simulink model "r2_b16a4x64f"  (R2012b)
settings: Solver=VariableStepDiscrete  SolverMode=SingleTasking  StartTime=0.0  StopTime=1  RelTol=1e-3
undefined symbols (not defined in the file): fft_stages, n_bits_ants, n_bits_xengs
libraries: xbsIndex_r4 x26846, casper_library_misc x230, xbsReplacements_r4 x24, casper_library_delays x8, xps_library x5, casper_library_communications x4
(part 19 of 227)

== system r2_b16a4x64f/status2 ==
  out_gbe_down : Inport
  out_rx_dest_err : Inport  Port=2
  out_feng_rx_err : Inport  Port=3
  out_fft_err : Inport  Port=4
  out_feng_qdr_err : Inport  Port=5
  out_feng_chk_err : Inport  Port=6
  out_adc_over : Inport  Port=7
  out_noise_diode_en : Inport  Port=8
  out_vacc_err : Inport  Port=9
  out_rx_bad_pkt : Inport  Port=10
  out_rx_bad_frame : Inport  Port=11
  out_tx_over : Inport  Port=12
  out_xeng_bad_dat : Inport  Port=13
  out_pack_err : Inport  Port=14
  out_rxing_data : Inport  Port=15
  out_txing_data : Inport  Port=16
  out_flushed : Inport  Port=17
  assert_adc_over : xbsIndex_r4/Assert  assert_type=on  type_source=Explicitly  gui_display_data_type=Boolean  arith_type=Boolean  n_bits=1  bin_pt=0  preci_type=Single  exp_width=8  frac_width=24  assert_rate=off  rate_source=Explicitly  period=1  output_port=on  block_type=assert
  assert_feng_chk_err : xbsIndex_r4/Assert  assert_type=on  type_source=Explicitly  gui_display_data_type=Boolean  arith_type=Boolean  n_bits=1  bin_pt=0  preci_type=Single  exp_width=8  frac_width=24  assert_rate=off  rate_source=Explicitly  period=1  output_port=on  block_type=assert
  assert_feng_qdr_err : xbsIndex_r4/Assert  assert_type=on  type_source=Explicitly  gui_display_data_type=Boolean  arith_type=Boolean  n_bits=1  bin_pt=0  preci_type=Single  exp_width=8  frac_width=24  assert_rate=off  rate_source=Explicitly  period=1  output_port=on  block_type=assert
  assert_feng_rx_err : xbsIndex_r4/Assert  assert_type=on  type_source=Explicitly  gui_display_data_type=Boolean  arith_type=Boolean  n_bits=1  bin_pt=0  preci_type=Single  exp_width=8  frac_width=24  assert_rate=off  rate_source=Explicitly  period=1  output_port=on  block_type=assert
  assert_fft_err : xbsIndex_r4/Assert  assert_type=on  type_source=Explicitly  gui_display_data_type=Boolean  arith_type=Boolean  n_bits=1  bin_pt=0  preci_type=Single  exp_width=8  frac_width=24  assert_rate=off  rate_source=Explicitly  period=1  output_port=on  block_type=assert
  assert_flushed : xbsIndex_r4/Assert  assert_type=on  type_source=Explicitly  gui_display_data_type=Boolean  arith_type=Boolean  n_bits=1  bin_pt=0  preci_type=Single  exp_width=8  frac_width=24  assert_rate=off  rate_source=Explicitly  period=1  output_port=on  block_type=assert
  assert_gbe_down : xbsIndex_r4/Assert  assert_type=on  type_source=Explicitly  gui_display_data_type=Boolean  arith_type=Boolean  n_bits=1  bin_pt=0  preci_type=Single  exp_width=8  frac_width=24  assert_rate=off  rate_source=Explicitly  period=1  output_port=on  block_type=assert
  assert_noise_diode_en : xbsIndex_r4/Assert  assert_type=on  type_source=Explicitly  gui_display_data_type=Boolean  arith_type=Boolean  n_bits=1  bin_pt=0  preci_type=Single  exp_width=8  frac_width=24  assert_rate=off  rate_source=Explicitly  period=1  output_port=on  block_type=assert
  assert_pack_err : xbsIndex_r4/Assert  assert_type=on  type_source=Explicitly  gui_display_data_type=Boolean  arith_type=Boolean  n_bits=1  bin_pt=0  preci_type=Single  exp_width=8  frac_width=24  assert_rate=off  rate_source=Explicitly  period=1  output_port=on  block_type=assert
  assert_rx_bad_frame : xbsIndex_r4/Assert  assert_type=on  type_source=Explicitly  gui_display_data_type=Boolean  arith_type=Boolean  n_bits=1  bin_pt=0  preci_type=Single  exp_width=8  frac_width=24  assert_rate=off  rate_source=Explicitly  period=1  output_port=on  block_type=assert
  assert_rx_bad_pkt : xbsIndex_r4/Assert  assert_type=on  type_source=Explicitly  gui_display_data_type=Boolean  arith_type=Boolean  n_bits=1  bin_pt=0  preci_type=Single  exp_width=8  frac_width=24  assert_rate=off  rate_source=Explicitly  period=1  output_port=on  block_type=assert
  assert_rx_dest_err : xbsIndex_r4/Assert  assert_type=on  type_source=Explicitly  gui_display_data_type=Boolean  arith_type=Boolean  n_bits=1  bin_pt=0  preci_type=Single  exp_width=8  frac_width=24  assert_rate=off  rate_source=Explicitly  period=1  output_port=on  block_type=assert
  assert_rxing_data : xbsIndex_r4/Assert  assert_type=on  type_source=Explicitly  gui_display_data_type=Boolean  arith_type=Boolean  n_bits=1  bin_pt=0  preci_type=Single  exp_width=8  frac_width=24  assert_rate=off  rate_source=Explicitly  period=1  output_port=on  block_type=assert
  assert_tx_over : xbsIndex_r4/Assert  assert_type=on  type_source=Explicitly  gui_display_data_type=Boolean  arith_type=Boolean  n_bits=1  bin_pt=0  preci_type=Single  exp_width=8  frac_width=24  assert_rate=off  rate_source=Explicitly  period=1  output_port=on  block_type=assert
  assert_txing_data : xbsIndex_r4/Assert  assert_type=on  type_source=Explicitly  gui_display_data_type=Boolean  arith_type=Boolean  n_bits=1  bin_pt=0  preci_type=Single  exp_width=8  frac_width=24  assert_rate=off  rate_source=Explicitly  period=1  output_port=on  block_type=assert
  assert_vacc_err : xbsIndex_r4/Assert  assert_type=on  type_source=Explicitly  gui_display_data_type=Boolean  arith_type=Boolean  n_bits=1  bin_pt=0  preci_type=Single  exp_width=8  frac_width=24  assert_rate=off  rate_source=Explicitly  period=1  output_port=on  block_type=assert
  assert_xeng_bad_dat : xbsIndex_r4/Assert  assert_type=on  type_source=Explicitly  gui_display_data_type=Boolean  arith_type=Boolean  n_bits=1  bin_pt=0  preci_type=Single  exp_width=8  frac_width=24  assert_rate=off  rate_source=Explicitly  period=1  output_port=on  block_type=assert
  cast_gw : xbsIndex_r4/Convert  gui_display_data_type=Fixed-point  arith_type=Unsigned  n_bits=32  bin_pt=0  float_type=Single  exp_bits=8  fraction_bits=24  quantization=Truncate  overflow=Wrap  en=off  latency=0  dbl_ovrd=off  pipeline=off  block_type=convert
  concatenate : xbsIndex_r4/Concat  num_inputs=17  dbl_ovrd=off  block_type=concat
  io_delay : xbsIndex_r4/Delay  rst=off  infoeditControl=Selection of Reset will increase slice count due to use of real FFs and instead of SRLs  en=off  latency=2  dbl_ovrd=off  reg_retiming=on  block_type=delay
  r2_b16a4x64f_status2_user_data_in : xbsIndex_r4/Gateway Out  inherit_from_input=off  hdl_port=on  timing_constraint=None  locs_specified=off  LOCs={}  UseAsDAC=off  DACChannel='1'  block_type=gatewayout
  reint{1..17} (17 alike) : xbsIndex_r4/Reinterpret  force_arith_type=on  arith_type=Unsigned  force_bin_pt=on  bin_pt=0  block_type=reinterpret
  sim_out : Terminator
  wires:
  concatenate/1 -> io_delay/1
  io_delay/1 -> cast_gw/1
  cast_gw/1 -> r2_b16a4x64f_status2_user_data_in/1
  r2_b16a4x64f_status2_user_data_in/1 -> sim_out/1
  out_gbe_down/1 -> assert_gbe_down/1
  assert_gbe_down/1 -> reint1/1
  reint1/1 -> concatenate/1
  out_rx_dest_err/1 -> assert_rx_dest_err/1
  assert_rx_dest_err/1 -> reint2/1
  reint2/1 -> concatenate/2
  out_feng_rx_err/1 -> assert_feng_rx_err/1
  assert_feng_rx_err/1 -> reint3/1
  reint3/1 -> concatenate/3
  out_fft_err/1 -> assert_fft_err/1
  assert_fft_err/1 -> reint4/1
  reint4/1 -> concatenate/4
  out_feng_qdr_err/1 -> assert_feng_qdr_err/1
  assert_feng_qdr_err/1 -> reint5/1
  reint5/1 -> concatenate/5
  out_feng_chk_err/1 -> assert_feng_chk_err/1
  assert_feng_chk_err/1 -> reint6/1
  reint6/1 -> concatenate/6
  out_adc_over/1 -> assert_adc_over/1
  assert_adc_over/1 -> reint7/1
  reint7/1 -> concatenate/7
  out_noise_diode_en/1 -> assert_noise_diode_en/1
  assert_noise_diode_en/1 -> reint8/1
  reint8/1 -> concatenate/8
  out_vacc_err/1 -> assert_vacc_err/1
  assert_vacc_err/1 -> reint9/1
  reint9/1 -> concatenate/9
  out_rx_bad_pkt/1 -> assert_rx_bad_pkt/1
  assert_rx_bad_pkt/1 -> reint10/1
  reint10/1 -> concatenate/10
  out_rx_bad_frame/1 -> assert_rx_bad_frame/1
  assert_rx_bad_frame/1 -> reint11/1
  reint11/1 -> concatenate/11
  out_tx_over/1 -> assert_tx_over/1
  assert_tx_over/1 -> reint12/1
  reint12/1 -> concatenate/12
  out_xeng_bad_dat/1 -> assert_xeng_bad_dat/1
  assert_xeng_bad_dat/1 -> reint13/1
  reint13/1 -> concatenate/13
  out_pack_err/1 -> assert_pack_err/1
  assert_pack_err/1 -> reint14/1
  reint14/1 -> concatenate/14
  out_rxing_data/1 -> assert_rxing_data/1
  assert_rxing_data/1 -> reint15/1
  reint15/1 -> concatenate/15
  out_txing_data/1 -> assert_txing_data/1
  assert_txing_data/1 -> reint16/1
  reint16/1 -> concatenate/16
  out_flushed/1 -> assert_flushed/1
  assert_flushed/1 -> reint17/1
  reint17/1 -> concatenate/17

== system r2_b16a4x64f/status3 ==
  out_gbe_down : Inport
  out_rx_dest_err : Inport  Port=2
  out_feng_rx_err : Inport  Port=3
  out_fft_err : Inport  Port=4
  out_feng_qdr_err : Inport  Port=5
  out_feng_chk_err : Inport  Port=6
  out_adc_over : Inport  Port=7
  out_noise_diode_en : Inport  Port=8
  out_vacc_err : Inport  Port=9
  out_rx_bad_pkt : Inport  Port=10
  out_rx_bad_frame : Inport  Port=11
  out_tx_over : Inport  Port=12
  out_xeng_bad_dat : Inport  Port=13
  out_pack_err : Inport  Port=14
  out_rxing_data : Inport  Port=15
  out_txing_data : Inport  Port=16
  out_flushed : Inport  Port=17
  assert_adc_over : xbsIndex_r4/Assert  assert_type=on  type_source=Explicitly  gui_display_data_type=Boolean  arith_type=Boolean  n_bits=1  bin_pt=0  preci_type=Single  exp_width=8  frac_width=24  assert_rate=off  rate_source=Explicitly  period=1  output_port=on  block_type=assert
  assert_feng_chk_err : xbsIndex_r4/Assert  assert_type=on  type_source=Explicitly  gui_display_data_type=Boolean  arith_type=Boolean  n_bits=1  bin_pt=0  preci_type=Single  exp_width=8  frac_width=24  assert_rate=off  rate_source=Explicitly  period=1  output_port=on  block_type=assert
  assert_feng_qdr_err : xbsIndex_r4/Assert  assert_type=on  type_source=Explicitly  gui_display_data_type=Boolean  arith_type=Boolean  n_bits=1  bin_pt=0  preci_type=Single  exp_width=8  frac_width=24  assert_rate=off  rate_source=Explicitly  period=1  output_port=on  block_type=assert
  assert_feng_rx_err : xbsIndex_r4/Assert  assert_type=on  type_source=Explicitly  gui_display_data_type=Boolean  arith_type=Boolean  n_bits=1  bin_pt=0  preci_type=Single  exp_width=8  frac_width=24  assert_rate=off  rate_source=Explicitly  period=1  output_port=on  block_type=assert
  assert_fft_err : xbsIndex_r4/Assert  assert_type=on  type_source=Explicitly  gui_display_data_type=Boolean  arith_type=Boolean  n_bits=1  bin_pt=0  preci_type=Single  exp_width=8  frac_width=24  assert_rate=off  rate_source=Explicitly  period=1  output_port=on  block_type=assert
  assert_flushed : xbsIndex_r4/Assert  assert_type=on  type_source=Explicitly  gui_display_data_type=Boolean  arith_type=Boolean  n_bits=1  bin_pt=0  preci_type=Single  exp_width=8  frac_width=24  assert_rate=off  rate_source=Explicitly  period=1  output_port=on  block_type=assert
  assert_gbe_down : xbsIndex_r4/Assert  assert_type=on  type_source=Explicitly  gui_display_data_type=Boolean  arith_type=Boolean  n_bits=1  bin_pt=0  preci_type=Single  exp_width=8  frac_width=24  assert_rate=off  rate_source=Explicitly  period=1  output_port=on  block_type=assert
  assert_noise_diode_en : xbsIndex_r4/Assert  assert_type=on  type_source=Explicitly  gui_display_data_type=Boolean  arith_type=Boolean  n_bits=1  bin_pt=0  preci_type=Single  exp_width=8  frac_width=24  assert_rate=off  rate_source=Explicitly  period=1  output_port=on  block_type=assert
  assert_pack_err : xbsIndex_r4/Assert  assert_type=on  type_source=Explicitly  gui_display_data_type=Boolean  arith_type=Boolean  n_bits=1  bin_pt=0  preci_type=Single  exp_width=8  frac_width=24  assert_rate=off  rate_source=Explicitly  period=1  output_port=on  block_type=assert
  assert_rx_bad_frame : xbsIndex_r4/Assert  assert_type=on  type_source=Explicitly  gui_display_data_type=Boolean  arith_type=Boolean  n_bits=1  bin_pt=0  preci_type=Single  exp_width=8  frac_width=24  assert_rate=off  rate_source=Explicitly  period=1  output_port=on  block_type=assert
  assert_rx_bad_pkt : xbsIndex_r4/Assert  assert_type=on  type_source=Explicitly  gui_display_data_type=Boolean  arith_type=Boolean  n_bits=1  bin_pt=0  preci_type=Single  exp_width=8  frac_width=24  assert_rate=off  rate_source=Explicitly  period=1  output_port=on  block_type=assert
  assert_rx_dest_err : xbsIndex_r4/Assert  assert_type=on  type_source=Explicitly  gui_display_data_type=Boolean  arith_type=Boolean  n_bits=1  bin_pt=0  preci_type=Single  exp_width=8  frac_width=24  assert_rate=off  rate_source=Explicitly  period=1  output_port=on  block_type=assert
  assert_rxing_data : xbsIndex_r4/Assert  assert_type=on  type_source=Explicitly  gui_display_data_type=Boolean  arith_type=Boolean  n_bits=1  bin_pt=0  preci_type=Single  exp_width=8  frac_width=24  assert_rate=off  rate_source=Explicitly  period=1  output_port=on  block_type=assert
  assert_tx_over : xbsIndex_r4/Assert  assert_type=on  type_source=Explicitly  gui_display_data_type=Boolean  arith_type=Boolean  n_bits=1  bin_pt=0  preci_type=Single  exp_width=8  frac_width=24  assert_rate=off  rate_source=Explicitly  period=1  output_port=on  block_type=assert
  assert_txing_data : xbsIndex_r4/Assert  assert_type=on  type_source=Explicitly  gui_display_data_type=Boolean  arith_type=Boolean  n_bits=1  bin_pt=0  preci_type=Single  exp_width=8  frac_width=24  assert_rate=off  rate_source=Explicitly  period=1  output_port=on  block_type=assert
  assert_vacc_err : xbsIndex_r4/Assert  assert_type=on  type_source=Explicitly  gui_display_data_type=Boolean  arith_type=Boolean  n_bits=1  bin_pt=0  preci_type=Single  exp_width=8  frac_width=24  assert_rate=off  rate_source=Explicitly  period=1  output_port=on  block_type=assert
  assert_xeng_bad_dat : xbsIndex_r4/Assert  assert_type=on  type_source=Explicitly  gui_display_data_type=Boolean  arith_type=Boolean  n_bits=1  bin_pt=0  preci_type=Single  exp_width=8  frac_width=24  assert_rate=off  rate_source=Explicitly  period=1  output_port=on  block_type=assert
  cast_gw : xbsIndex_r4/Convert  gui_display_data_type=Fixed-point  arith_type=Unsigned  n_bits=32  bin_pt=0  float_type=Single  exp_bits=8  fraction_bits=24  quantization=Truncate  overflow=Wrap  en=off  latency=0  dbl_ovrd=off  pipeline=off  block_type=convert
  concatenate : xbsIndex_r4/Concat  num_inputs=17  dbl_ovrd=off  block_type=concat
  io_delay : xbsIndex_r4/Delay  rst=off  infoeditControl=Selection of Reset will increase slice count due to use of real FFs and instead of SRLs  en=off  latency=2  dbl_ovrd=off  reg_retiming=on  block_type=delay
  r2_b16a4x64f_status3_user_data_in : xbsIndex_r4/Gateway Out  inherit_from_input=off  hdl_port=on  timing_constraint=None  locs_specified=off  LOCs={}  UseAsDAC=off  DACChannel='1'  block_type=gatewayout
  reint{1..17} (17 alike) : xbsIndex_r4/Reinterpret  force_arith_type=on  arith_type=Unsigned  force_bin_pt=on  bin_pt=0  block_type=reinterpret
  sim_out : Terminator
  wires:
  concatenate/1 -> io_delay/1
  io_delay/1 -> cast_gw/1
  cast_gw/1 -> r2_b16a4x64f_status3_user_data_in/1
  r2_b16a4x64f_status3_user_data_in/1 -> sim_out/1
  out_gbe_down/1 -> assert_gbe_down/1
  assert_gbe_down/1 -> reint1/1
  reint1/1 -> concatenate/1
  out_rx_dest_err/1 -> assert_rx_dest_err/1
  assert_rx_dest_err/1 -> reint2/1
  reint2/1 -> concatenate/2
  out_feng_rx_err/1 -> assert_feng_rx_err/1
  assert_feng_rx_err/1 -> reint3/1
  reint3/1 -> concatenate/3
  out_fft_err/1 -> assert_fft_err/1
  assert_fft_err/1 -> reint4/1
  reint4/1 -> concatenate/4
  out_feng_qdr_err/1 -> assert_feng_qdr_err/1
  assert_feng_qdr_err/1 -> reint5/1
  reint5/1 -> concatenate/5
  out_feng_chk_err/1 -> assert_feng_chk_err/1
  assert_feng_chk_err/1 -> reint6/1
  reint6/1 -> concatenate/6
  out_adc_over/1 -> assert_adc_over/1
  assert_adc_over/1 -> reint7/1
  reint7/1 -> concatenate/7
  out_noise_diode_en/1 -> assert_noise_diode_en/1
  assert_noise_diode_en/1 -> reint8/1
  reint8/1 -> concatenate/8
  out_vacc_err/1 -> assert_vacc_err/1
  assert_vacc_err/1 -> reint9/1
  reint9/1 -> concatenate/9
  out_rx_bad_pkt/1 -> assert_rx_bad_pkt/1
  assert_rx_bad_pkt/1 -> reint10/1
  reint10/1 -> concatenate/10
  out_rx_bad_frame/1 -> assert_rx_bad_frame/1
  assert_rx_bad_frame/1 -> reint11/1
  reint11/1 -> concatenate/11
  out_tx_over/1 -> assert_tx_over/1
  assert_tx_over/1 -> reint12/1
  reint12/1 -> concatenate/12
  out_xeng_bad_dat/1 -> assert_xeng_bad_dat/1
  assert_xeng_bad_dat/1 -> reint13/1
  reint13/1 -> concatenate/13
  out_pack_err/1 -> assert_pack_err/1
  assert_pack_err/1 -> reint14/1
  reint14/1 -> concatenate/14
  out_rxing_data/1 -> assert_rxing_data/1
  assert_rxing_data/1 -> reint15/1
  reint15/1 -> concatenate/15
  out_txing_data/1 -> assert_txing_data/1
  assert_txing_data/1 -> reint16/1
  reint16/1 -> concatenate/16
  out_flushed/1 -> assert_flushed/1
  assert_flushed/1 -> reint17/1
  reint17/1 -> concatenate/17
